simulink model "Cell_Balancer_V_2"  (R2026b)
settings: Solver=VariableStepAuto  StopTime=72000
InitFcn:
  | R=4.2
  | A=.2
  | B=.25
  | C=.24
  | D=.23
  | E=.29
  | F=.22
  | G=.26
  | H=.27
  | I=.28
  | J=.21
libraries: fl_lib x43, nesl_utility x33, batt_lib x10, BatteryCurrentManagement x1
(part 1 of 4)
settings Model: Creator=cbast  LastModifiedBy=cbast
settings SimscapeCC: SimscapeLogType=all  SimscapeNominalValues="[{\"value\":\"1\",\"unit\":\"A\"},{\"value\":\"1\",\"unit\":\"bar\"},{\"value\":\"1\",\"unit\":\"cm^2\"},{\"value\":\"1\",\"unit\":\"cm^3/s\"},{\"value\":\"1\",\"unit\":\"kJ/kg\"},{\"value\":\"1\",\"unit\":\"kW\"},{\"value\":\"1\",\"unit\":\"l\"},{\"value\":\"1\",\"unit\":\"N\"},{\"value\":\"1\",\"unit\":\"N*m\"},{\"value\":\"1\",\"unit\":\"V\"},{\"value\":\"0.001\",\"unit\":\"Wb\"}]"  SimscapeUseEnergyAccounting=off

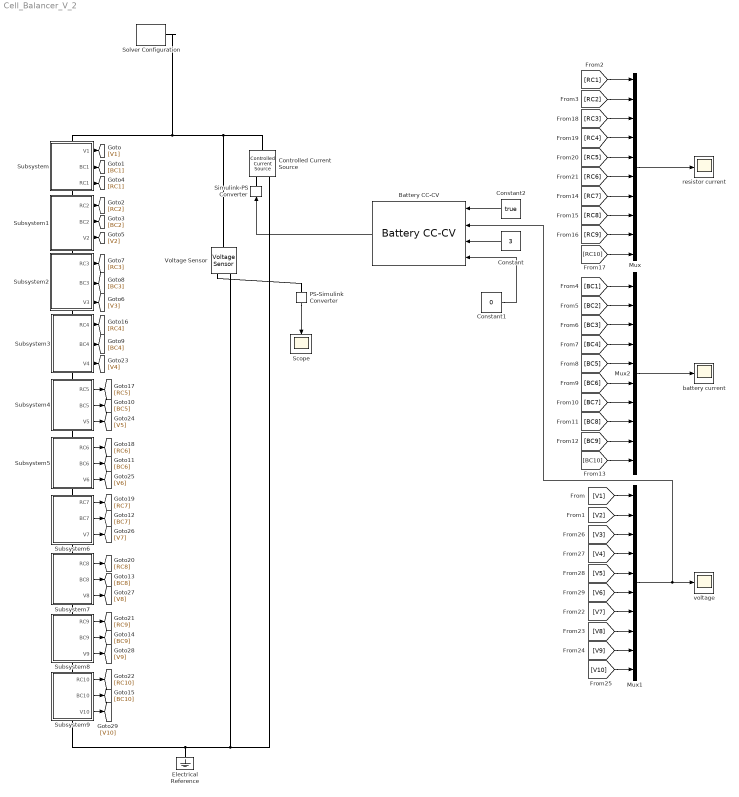
== system Cell_Balancer_V_2 ==
  Battery CC-CV : BatteryCurrentManagement/Battery CC-CV  MinMaxFlag=off  MaxCellVoltage=4.2  Kp=100  Ki=10  Kaw=1  Kt=1  Ts=.1
      settings: LibrarySourceBlock=batt_sl_lib/Current Management/Battery CC-CV
  Constant : Constant  Value=3
  Constant1 : Constant  Value=0
  Constant2 : Constant  Value=true  OutDataTypeStr=boolean
  Controlled Current Source : fl_lib/Electrical/Electrical Sources/Controlled Current Source
  Electrical Reference : fl_lib/Electrical/Electrical Elements/Electrical Reference
  Mux : Mux  Inputs=10
  Mux1 : Mux  Inputs=10
  Mux2 : Mux  Inputs=10
  PS-Simulink Converter : nesl_utility/PS-Simulink Converter  PhysicalDomain=network_engine_domain  SubClassName=ps_output  LeftPortType=input  RightPortType=output  PseudoPeriodic=off  Frequencies=[]  VectorFormat=inherit  Unit=inherit  AffineConversion=off
  Scope : Scope
      settings: ActiveDisplayYMinimum=29.7505090759505  ActiveDisplayYMaximum=43.345712012643816  DataLoggingVariableName=ScopeData3
  Simulink-PS Converter : nesl_utility/Simulink-PS Converter  PhysicalDomain=network_engine_domain  SubClassName=ps_input  LeftPortType=input  RightPortType=output  PseudoPeriodic=off  Frequencies=[]  NoiseDistribution=none  NoiseParameters=[]  Unit=A  AffineConversion=off  FilteringAndDerivatives=provide  SimscapeFilterOrder=1  InputFilterTimeConstant=0.001  UdotUserProvided=0
  Solver Configuration : nesl_utility/Solver Configuration  PhysicalDomain=network_engine_domain  SubClassName=solver  LeftPortType=input  RightPortType=generic  Tones=[]  Harmonics=[]  SimulateNoise=off  Profile=off  UseLocalSampling=off  EnableSwitchedLinearOptims=on  FrequencyDomain=off  UseCCode=off  RelTol=0.001  AbsTol=0.001  MinStep=1e-09  ToWorkspace=off  RevertToSquareIcSolve=off  NumHomotopyIterations=100  PhasorMode=off  PhasorModeNumHarmonics=1  ConsistencySolver=NEWTON_XTOL_AFTER_FTOL  CanonicalOrdering=CANONICAL  OptimizeIntermediates=OPTIMIZED  MulticoreSolverChoice=BACKWARD_EULER  IndexReductionMethod=DerivativeReplacement  DoDC=off  ResidualTolerance=1e-09  ConsistencyTolSource=GLOBAL  ConsistencyAbsTol=0.001  ConsistencyRelTol=0.001  ConsistencyTolFactor=0.001  UseLocalSolver=off  LocalSolverChoice=NE_BACKWARD_EULER_ADVANCER  ResolveIndetEquations=on  FunctionEvalNumThread=1  LocalSolverSampleTime=0.001  DoFixedCost=off  MaxNonlinIter=3  MaxModeIter=2  ComputeImpulses=off  ImpulseIterations=2  LinearAlgebra=auto  LinearAlgebraNumThread=0  EquationFormulation=NE_TIME_EF  DelaysMemoryBudget=1024  AutomaticFiltering=on  FilteringTimeConstant=0.001  PartitionStorageMethod=AS_NEEDED  PartitionMemoryBudget=1024  PartitionMethod=BALANCED  MultibodyUseLocalSolver=off  MultibodyLocalSolverChoice=ODE1  MultibodyLocalSolverSampleTime=0.001
  Subsystem : Subsystem
      settings: PortSchema="{\"entries\":[{\"content\":{\"sides\":[{\"content\":{\"connectorIds\":[\"LConn1\"]},\"type\":\"ConnectorPlacement.EquallySpacedRectSide\",\"uuid\":\"cf979a16-a91b-4829-8e8c-47878ae37a6b\"},{\"content\":{\"connectorIds\":[\"Out1\",\"Out2\",\"Out3\"],\"side\":\"RIGHT\"},\"type\":\"ConnectorPlacement.EquallySpacedRectSide\",\"uuid\":\"6e20e9dd-b02d-4dd9-9bba-83c5ab962d64\"},{\"content\":{\"connectorIds\":[\"LConn2\"],\"side\":\"TOP\"},\"type\":\"ConnectorPlacement.EquallySpacedRectSide\",\"uuid\":\"a7acf913-948b-411d-bbec-040cc670f398\"},{\"content\":{\"connectorIds\":[\"RConn1\"],\"side\":\"BOTTOM\"},\"type\":\"ConnectorPlacement.EquallySpacedRectSide\",\"uuid\":\"1d5d0df0-1bd4-46ff-b3f2-dbc3a67d8787\"}]},\"type\":\"ConnectorPlacement.EquallySpacedConnector\",\"uuid\":\"c3ff8ae8-2df9-499f-8763-7ecb3999170d\"}],\"packageUris\":[\"http://schema.mathworks.com/mf0/Connector/R2020b\"],\"version\":\"1.0\"}"
  Subsystem1 : Subsystem
      settings: PortSchema="{\"entries\":[{\"content\":{\"sides\":[{\"content\":{\"connectorIds\":[\"LConn1\"]},\"type\":\"ConnectorPlacement.EquallySpacedRectSide\",\"uuid\":\"b864f2b2-5928-4e80-8598-6ae066b8b686\"},{\"content\":{\"connectorIds\":[\"Out1\",\"Out2\",\"Out3\"],\"side\":\"RIGHT\"},\"type\":\"ConnectorPlacement.EquallySpacedRectSide\",\"uuid\":\"4c0824a7-ad18-427d-825c-0601e9e3c2a5\"},{\"content\":{\"connectorIds\":[\"LConn2\"],\"side\":\"TOP\"},\"type\":\"ConnectorPlacement.EquallySpacedRectSide\",\"uuid\":\"58eac08c-ab90-4096-8c71-26645031beff\"},{\"content\":{\"connectorIds\":[\"RConn1\"],\"side\":\"BOTTOM\"},\"type\":\"ConnectorPlacement.EquallySpacedRectSide\",\"uuid\":\"928b4b2b-69e3-456a-8822-74aa848d5ef0\"}]},\"type\":\"ConnectorPlacement.EquallySpacedConnector\",\"uuid\":\"d1889de4-d401-4a0f-84af-d9f011bf39d7\"}],\"packageUris\":[\"http://schema.mathworks.com/mf0/Connector/R2020b\"],\"version\":\"1.0\"}"
  Subsystem2 : Subsystem
      settings: PortSchema="{\"entries\":[{\"content\":{\"sides\":[{\"content\":{\"connectorIds\":[\"LConn1\"]},\"type\":\"ConnectorPlacement.EquallySpacedRectSide\",\"uuid\":\"b864f2b2-5928-4e80-8598-6ae066b8b686\"},{\"content\":{\"connectorIds\":[\"Out1\",\"Out2\",\"Out3\"],\"side\":\"RIGHT\"},\"type\":\"ConnectorPlacement.EquallySpacedRectSide\",\"uuid\":\"4c0824a7-ad18-427d-825c-0601e9e3c2a5\"},{\"content\":{\"connectorIds\":[\"LConn2\"],\"side\":\"TOP\"},\"type\":\"ConnectorPlacement.EquallySpacedRectSide\",\"uuid\":\"58eac08c-ab90-4096-8c71-26645031beff\"},{\"content\":{\"connectorIds\":[\"RConn1\"],\"side\":\"BOTTOM\"},\"type\":\"ConnectorPlacement.EquallySpacedRectSide\",\"uuid\":\"928b4b2b-69e3-456a-8822-74aa848d5ef0\"}]},\"type\":\"ConnectorPlacement.EquallySpacedConnector\",\"uuid\":\"d1889de4-d401-4a0f-84af-d9f011bf39d7\"}],\"packageUris\":[\"http://schema.mathworks.com/mf0/Connector/R2020b\"],\"version\":\"1.0\"}"
  Subsystem3 : Subsystem
      settings: PortSchema="{\"entries\":[{\"content\":{\"sides\":[{\"content\":{\"connectorIds\":[\"LConn1\"]},\"type\":\"ConnectorPlacement.EquallySpacedRectSide\",\"uuid\":\"b864f2b2-5928-4e80-8598-6ae066b8b686\"},{\"content\":{\"connectorIds\":[\"Out1\",\"Out2\",\"Out3\"],\"side\":\"RIGHT\"},\"type\":\"ConnectorPlacement.EquallySpacedRectSide\",\"uuid\":\"4c0824a7-ad18-427d-825c-0601e9e3c2a5\"},{\"content\":{\"connectorIds\":[\"LConn2\"],\"side\":\"TOP\"},\"type\":\"ConnectorPlacement.EquallySpacedRectSide\",\"uuid\":\"58eac08c-ab90-4096-8c71-26645031beff\"},{\"content\":{\"connectorIds\":[\"RConn1\"],\"side\":\"BOTTOM\"},\"type\":\"ConnectorPlacement.EquallySpacedRectSide\",\"uuid\":\"928b4b2b-69e3-456a-8822-74aa848d5ef0\"}]},\"type\":\"ConnectorPlacement.EquallySpacedConnector\",\"uuid\":\"d1889de4-d401-4a0f-84af-d9f011bf39d7\"}],\"packageUris\":[\"http://schema.mathworks.com/mf0/Connector/R2020b\"],\"version\":\"1.0\"}"
  Subsystem4 : Subsystem
      settings: PortSchema="{\"entries\":[{\"content\":{\"sides\":[{\"content\":{\"connectorIds\":[\"LConn1\"]},\"type\":\"ConnectorPlacement.EquallySpacedRectSide\",\"uuid\":\"b864f2b2-5928-4e80-8598-6ae066b8b686\"},{\"content\":{\"connectorIds\":[\"Out1\",\"Out2\",\"Out3\"],\"side\":\"RIGHT\"},\"type\":\"ConnectorPlacement.EquallySpacedRectSide\",\"uuid\":\"4c0824a7-ad18-427d-825c-0601e9e3c2a5\"},{\"content\":{\"connectorIds\":[\"LConn2\"],\"side\":\"TOP\"},\"type\":\"ConnectorPlacement.EquallySpacedRectSide\",\"uuid\":\"58eac08c-ab90-4096-8c71-26645031beff\"},{\"content\":{\"connectorIds\":[\"RConn1\"],\"side\":\"BOTTOM\"},\"type\":\"ConnectorPlacement.EquallySpacedRectSide\",\"uuid\":\"928b4b2b-69e3-456a-8822-74aa848d5ef0\"}]},\"type\":\"ConnectorPlacement.EquallySpacedConnector\",\"uuid\":\"d1889de4-d401-4a0f-84af-d9f011bf39d7\"}],\"packageUris\":[\"http://schema.mathworks.com/mf0/Connector/R2020b\"],\"version\":\"1.0\"}"
  Subsystem5 : Subsystem
      settings: PortSchema="{\"entries\":[{\"content\":{\"sides\":[{\"content\":{\"connectorIds\":[\"LConn1\"]},\"type\":\"ConnectorPlacement.EquallySpacedRectSide\",\"uuid\":\"b864f2b2-5928-4e80-8598-6ae066b8b686\"},{\"content\":{\"connectorIds\":[\"Out1\",\"Out2\",\"Out3\"],\"side\":\"RIGHT\"},\"type\":\"ConnectorPlacement.EquallySpacedRectSide\",\"uuid\":\"4c0824a7-ad18-427d-825c-0601e9e3c2a5\"},{\"content\":{\"connectorIds\":[\"LConn2\"],\"side\":\"TOP\"},\"type\":\"ConnectorPlacement.EquallySpacedRectSide\",\"uuid\":\"58eac08c-ab90-4096-8c71-26645031beff\"},{\"content\":{\"connectorIds\":[\"RConn1\"],\"side\":\"BOTTOM\"},\"type\":\"ConnectorPlacement.EquallySpacedRectSide\",\"uuid\":\"928b4b2b-69e3-456a-8822-74aa848d5ef0\"}]},\"type\":\"ConnectorPlacement.EquallySpacedConnector\",\"uuid\":\"d1889de4-d401-4a0f-84af-d9f011bf39d7\"}],\"packageUris\":[\"http://schema.mathworks.com/mf0/Connector/R2020b\"],\"version\":\"1.0\"}"
  Subsystem6 : Subsystem
      settings: PortSchema="{\"entries\":[{\"content\":{\"sides\":[{\"content\":{\"connectorIds\":[\"LConn1\"]},\"type\":\"ConnectorPlacement.EquallySpacedRectSide\",\"uuid\":\"b864f2b2-5928-4e80-8598-6ae066b8b686\"},{\"content\":{\"connectorIds\":[\"Out1\",\"Out2\",\"Out3\"],\"side\":\"RIGHT\"},\"type\":\"ConnectorPlacement.EquallySpacedRectSide\",\"uuid\":\"4c0824a7-ad18-427d-825c-0601e9e3c2a5\"},{\"content\":{\"connectorIds\":[\"LConn2\"],\"side\":\"TOP\"},\"type\":\"ConnectorPlacement.EquallySpacedRectSide\",\"uuid\":\"58eac08c-ab90-4096-8c71-26645031beff\"},{\"content\":{\"connectorIds\":[\"RConn1\"],\"side\":\"BOTTOM\"},\"type\":\"ConnectorPlacement.EquallySpacedRectSide\",\"uuid\":\"928b4b2b-69e3-456a-8822-74aa848d5ef0\"}]},\"type\":\"ConnectorPlacement.EquallySpacedConnector\",\"uuid\":\"d1889de4-d401-4a0f-84af-d9f011bf39d7\"}],\"packageUris\":[\"http://schema.mathworks.com/mf0/Connector/R2020b\"],\"version\":\"1.0\"}"
  Subsystem7 : Subsystem
      settings: PortSchema="{\"entries\":[{\"content\":{\"sides\":[{\"content\":{\"connectorIds\":[\"LConn1\"]},\"type\":\"ConnectorPlacement.EquallySpacedRectSide\",\"uuid\":\"b864f2b2-5928-4e80-8598-6ae066b8b686\"},{\"content\":{\"connectorIds\":[\"Out1\",\"Out2\",\"Out3\"],\"side\":\"RIGHT\"},\"type\":\"ConnectorPlacement.EquallySpacedRectSide\",\"uuid\":\"4c0824a7-ad18-427d-825c-0601e9e3c2a5\"},{\"content\":{\"connectorIds\":[\"LConn2\"],\"side\":\"TOP\"},\"type\":\"ConnectorPlacement.EquallySpacedRectSide\",\"uuid\":\"58eac08c-ab90-4096-8c71-26645031beff\"},{\"content\":{\"connectorIds\":[\"RConn1\"],\"side\":\"BOTTOM\"},\"type\":\"ConnectorPlacement.EquallySpacedRectSide\",\"uuid\":\"928b4b2b-69e3-456a-8822-74aa848d5ef0\"}]},\"type\":\"ConnectorPlacement.EquallySpacedConnector\",\"uuid\":\"d1889de4-d401-4a0f-84af-d9f011bf39d7\"}],\"packageUris\":[\"http://schema.mathworks.com/mf0/Connector/R2020b\"],\"version\":\"1.0\"}"
  Subsystem8 : Subsystem
      settings: PortSchema="{\"entries\":[{\"content\":{\"sides\":[{\"content\":{\"connectorIds\":[\"LConn1\"]},\"type\":\"ConnectorPlacement.EquallySpacedRectSide\",\"uuid\":\"b864f2b2-5928-4e80-8598-6ae066b8b686\"},{\"content\":{\"connectorIds\":[\"Out1\",\"Out2\",\"Out3\"],\"side\":\"RIGHT\"},\"type\":\"ConnectorPlacement.EquallySpacedRectSide\",\"uuid\":\"4c0824a7-ad18-427d-825c-0601e9e3c2a5\"},{\"content\":{\"connectorIds\":[\"LConn2\"],\"side\":\"TOP\"},\"type\":\"ConnectorPlacement.EquallySpacedRectSide\",\"uuid\":\"58eac08c-ab90-4096-8c71-26645031beff\"},{\"content\":{\"connectorIds\":[\"RConn1\"],\"side\":\"BOTTOM\"},\"type\":\"ConnectorPlacement.EquallySpacedRectSide\",\"uuid\":\"928b4b2b-69e3-456a-8822-74aa848d5ef0\"}]},\"type\":\"ConnectorPlacement.EquallySpacedConnector\",\"uuid\":\"d1889de4-d401-4a0f-84af-d9f011bf39d7\"}],\"packageUris\":[\"http://schema.mathworks.com/mf0/Connector/R2020b\"],\"version\":\"1.0\"}"
  Subsystem9 : Subsystem
      settings: PortSchema="{\"entries\":[{\"content\":{\"sides\":[{\"content\":{\"connectorIds\":[\"LConn1\"]},\"type\":\"ConnectorPlacement.EquallySpacedRectSide\",\"uuid\":\"b864f2b2-5928-4e80-8598-6ae066b8b686\"},{\"content\":{\"connectorIds\":[\"Out1\",\"Out2\",\"Out3\"],\"side\":\"RIGHT\"},\"type\":\"ConnectorPlacement.EquallySpacedRectSide\",\"uuid\":\"4c0824a7-ad18-427d-825c-0601e9e3c2a5\"},{\"content\":{\"connectorIds\":[\"LConn2\"],\"side\":\"TOP\"},\"type\":\"ConnectorPlacement.EquallySpacedRectSide\",\"uuid\":\"58eac08c-ab90-4096-8c71-26645031beff\"},{\"content\":{\"connectorIds\":[\"RConn1\"],\"side\":\"BOTTOM\"},\"type\":\"ConnectorPlacement.EquallySpacedRectSide\",\"uuid\":\"928b4b2b-69e3-456a-8822-74aa848d5ef0\"}]},\"type\":\"ConnectorPlacement.EquallySpacedConnector\",\"uuid\":\"d1889de4-d401-4a0f-84af-d9f011bf39d7\"}],\"packageUris\":[\"http://schema.mathworks.com/mf0/Connector/R2020b\"],\"version\":\"1.0\"}"
  Voltage Sensor : fl_lib/Electrical/Electrical Sensors/Voltage Sensor
  battery current : Scope
      settings: ActiveDisplayYMinimum=-0.32310664048068816  ActiveDisplayYMaximum=2.5809557460332671  DataLoggingVariableName=ScopeData2
  resistor current : Scope
      settings: ActiveDisplayYMinimum=0.68694599163620873  ActiveDisplayYMaximum=1.0369030277450046
  voltage : Scope
      settings: ActiveDisplayYMinimum=2.8851731648720769  ActiveDisplayYMaximum=4.3549927165290168
  wires:
  Mux/1 -> resistor current/1
  Mux1/1 -> Battery CC-CV/2, voltage/1
  [BC2] -> Mux2/2
  [BC1] -> Mux2/1
  Mux2/1 -> battery current/1
  [RC1] -> Mux/1
  [RC2] -> Mux/2
  [V2] -> Mux1/2
  [V1] -> Mux1/1
  Subsystem/1(V1) -> [V1]
  Subsystem/2(BC1) -> [BC1]
  Subsystem/3(RC1) -> [RC1]
  Subsystem1/1(RC2) -> [RC2]
  Subsystem1/2(BC2) -> [BC2]
  Subsystem1/3(V2) -> [V2]
  [BC3] -> Mux2/3
  [BC4] -> Mux2/4
  [BC5] -> Mux2/5
  [BC6] -> Mux2/6
  [BC7] -> Mux2/7
  [BC8] -> Mux2/8
  [BC9] -> Mux2/9
  [BC10] -> Mux2/10
  [RC5] -> Mux/5
  [RC4] -> Mux/4
  [RC6] -> Mux/6
  [RC10] -> Mux/10
  [RC9] -> Mux/9
  [RC8] -> Mux/8
  [RC7] -> Mux/7
  [V3] -> Mux1/3
  [V4] -> Mux1/4
  [V5] -> Mux1/5
  [V6] -> Mux1/6
  [V7] -> Mux1/7
  [V8] -> Mux1/8
  [V9] -> Mux1/9
  [V10] -> Mux1/10
  Subsystem2/3(V3) -> [V3]
  Subsystem2/2(BC3) -> [BC3]
  Subsystem2/1(RC3) -> [RC3]
  Subsystem3/2(BC4) -> [BC4]
  Subsystem5/2(BC6) -> [BC6]
  Subsystem3/1(RC4) -> [RC4]
  Subsystem4/1(RC5) -> [RC5]
  Subsystem4/2(BC5) -> [BC5]
  Subsystem3/3(V4) -> [V4]
  Subsystem4/3(V5) -> [V5]
  Subsystem5/1(RC6) -> [RC6]
  Subsystem5/3(V6) -> [V6]
  Subsystem6/1(RC7) -> [RC7]
  Subsystem6/2(BC7) -> [BC7]
  Subsystem7/3(V8) -> [V8]
  Subsystem8/3(V9) -> [V9]
  Subsystem7/2(BC8) -> [BC8]
  Subsystem7/1(RC8) -> [RC8]
  Subsystem6/3(V7) -> [V7]
  Subsystem8/1(RC9) -> [RC9]
  Subsystem8/2(BC9) -> [BC9]
  Subsystem9/1(RC10) -> [RC10]
  Subsystem9/2(BC10) -> [BC10]
  Subsystem9/3(V10) -> [V10]
  [RC3] -> Mux/3
  PS-Simulink Converter/1 -> Scope/1
  Battery CC-CV/1 -> Simulink-PS Converter/1
  Constant/1 -> Battery CC-CV/3
  Constant1/1 -> Battery CC-CV/4
  Constant2/1 -> Battery CC-CV/1
  connections:
  Simulink-PS Converter/RConn1 -- Controlled Current Source/RConn1
  Solver Configuration/RConn1 -- Controlled Current Source/LConn1 -- Voltage Sensor/LConn1 -- Subsystem/LConn2
  Controlled Current Source/RConn2 -- Subsystem9/RConn1 -- Electrical Reference/LConn1 -- Voltage Sensor/RConn2
  Subsystem/RConn1 -- Subsystem1/LConn2
  Subsystem2/LConn2 -- Subsystem1/RConn1
  Subsystem3/LConn2 -- Subsystem2/RConn1
  Subsystem4/LConn2 -- Subsystem3/RConn1
  Subsystem5/LConn2 -- Subsystem4/RConn1
  Subsystem6/LConn2 -- Subsystem5/RConn1
  Subsystem7/LConn2 -- Subsystem6/RConn1
  Subsystem8/LConn2 -- Subsystem7/RConn1
  Subsystem9/LConn2 -- Subsystem8/RConn1
  PS-Simulink Converter/LConn1 -- Voltage Sensor/RConn1

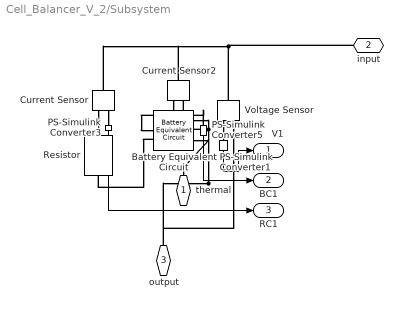
== system Cell_Balancer_V_2/Subsystem ==
  Battery Equivalent Circuit : batt_lib/Cells/Battery Equivalent Circuit  BatteryCapacity=3 A*hr  ThermalModel=simscape.battery.enum.cells.BatteryThermalModel.LumpedThermalMass  ExtrapolationMethod=simscape.enum.extrapolation.nearest  SOCBreakpoints=[0, .1, .25, .5, .75, .9, 1]  TemperatureBreakpoints=[278, 293, 313] K  OpenCircuitVoltage=[3.5057, 3.566, 3.6337, 3.7127, 3.9259, 4.0777, 4.1928] V  OpenCircuitVoltageThermal=|  VoltageRange=[0, inf] V  HysteresisModel=simscape.battery.enum.cells.HysteresisModel.none  MaximumHysteresisVoltage=[0, 0, 0, 0, 0, 0, 0] V  InstantaneousHysteresisVoltage=[0, 0, 0, 0, 0, 0, 0] V  HysteresisRate=0.1  MaximumHysteresisVoltageThermal=[0, 0, 0; 0, 0, 0; 0, 0, 0; 0, 0, 0; 0, 0, 0; 0, 0, 0; 0, 0, 0] V  InstantaneousHysteresisVoltageThermal=[0, 0, 0; 0, 0, 0; 0, 0, 0; 0, 0, 0; 0, 0, 0; 0, 0, 0; 0, 0, 0] V  HysteresisRateThermal=0.1  ResistanceSOCBreakpoints=[0, .1, .25, .5, .75, .9, 1]  ResistanceTemperatureBreakpoints=[278, 293, 313] K  ResistanceCurrentBreakpoints=[-1, 0, 1] A  CurrentDependence=simscape.battery.enum.cells.CurrentDependence.Disabled  R0=[.0085, .0085, .0087, .0082, .0083, .0085, .0085] Ohm  R0I=[.0117, .0085, .009; .011, .0085, .009; .0114, .0087, .0092; .0107, .0082, .0088; .0107, .0083, .0091; .0113, .0085, .0089; .0116, .0085, .0089] Ohm  R0Thermal=[.0117, .0085, .009; .011, .0085, .009; .0114, .0087, .0092; .0107, .0082, .0088; .0107, .0083, .0091; .0113, .0085, .0089; .0116, .0085, .0089] Ohm  R0ThermalI=repmat([.0117, .0085, .009; .011, .0085, .009; .0114, .0087, .0092; .0107, .0082, .0088; .0107, .0083, .0091; .0113, .0085, .0089; .0116, .0085, .0089], 1, 1, 3) Ohm  DischargeR0=[.0085, .0085, .0087, .0082, .0083, .0085, .0085] Ohm  ChargeR0=[.0085, .0085, .0087, .0082, .0083, .0085, .0085] Ohm  ChargeR0Thermal=[.0117, .0085, .009; .011, .0085, .009; .0114, .0087, .0092; .0107, .0082, .0088; .0107, .0083, .0091; .0113, .0085, .0089; .0116, .0085, .0089] Ohm  DischargeR0Thermal=[.0117, .0085, .009; .011, .0085, .009; .0114, .0087, .0092; .0107, .0082, .0088; .0107, .0083, .0091; .0113, .0085, .0089; .0116, .0085, .0089] Ohm  RCPairs=simscape.battery.enum.cells.RCPairs.noDynamics  R1=[.0029, .0024, .0026, .0016, .0023, .0018, .0017] Ohm  Tau1=[36, 45, 105, 29, 77, 33, 39] s  R2=[.0029, .0024, .0026, .0016, .0023, .0018, .0017] Ohm  Tau2=[36, 45, 105, 29, 77, 33, 39] s  R3=[.0029, .0024, .0026, .0016, .0023, .0018, .0017] Ohm  Tau3=[36, 45, 105, 29, 77, 33, 39] s  R1I=[.0109, .0029, .0013; .0069, .0024, .0012; .0047, .0026, .0013; .0034, .0016, .001; .0033, .0023, .0014; .0033, .0018, .0011; .0028, .0017, .0011] Ohm  Tau1I=[20, 36, 39; 31, 45, 39; 109, 105, 61; 36, 29, 26; 59, 77, 67; 40, 33, 29; 25, 39, 33] s  R2I=[.0109, .0029, .0013; .0069, .0024, .0012; .0047, .0026, .0013; .0034, .0016, .001; .0033, .0023, .0014; .0033, .0018, .0011; .0028, .0017, .0011] Ohm  Tau2I=[20, 36, 39; 31, 45, 39; 109, 105, 61; 36, 29, 26; 59, 77, 67; 40, 33, 29; 25, 39, 33] s  R3I=[.0109, .0029, .0013; .0069, .0024, .0012; .0047, .0026, .0013; .0034, .0016, .001; .0033, .0023, .0014; .0033, .0018, .0011; .0028, .0017, .0011] Ohm  Tau3I=[20, 36, 39; 31, 45, 39; 109, 105, 61; 36, 29, 26; 59, 77, 67; 40, 33, 29; 25, 39, 33] s  DischargeR1=[.0029, .0024, .0026, .0016, .0023, .0018, .0017] Ohm  DischargeTau1=[36, 45, 105, 29, 77, 33, 39] s  ChargeR1=[.0029, .0024, .0026, .0016, .0023, .0018, .0017] Ohm  ChargeTau1=[36, 45, 105, 29, 77, 33, 39] s  DischargeR2=[.0029, .0024, .0026, .0016, .0023, .0018, .0017] Ohm  DischargeTau2=[36, 45, 105, 29, 77, 33, 39] s  ChargeR2=[.0029, .0024, .0026, .0016, .0023, .0018, .0017] Ohm  ChargeTau2=[36, 45, 105, 29, 77, 33, 39] s  DischargeR3=[.0029, .0024, .0026, .0016, .0023, .0018, .0017] Ohm  DischargeTau3=[36, 45, 105, 29, 77, 33, 39] s  ChargeR3=[.0029, .0024, .0026, .0016, .0023, .0018, .0017] Ohm  ChargeTau3=[36, 45, 105, 29, 77, 33, 39] s  R1Thermal=[.0109, .0029, .0013; .0069, .0024, .0012; .0047, .0026, .0013; .0034, .0016, .001; .0033, .0023, .0014; .0033, .0018, .0011; .0028, .0017, .0011] Ohm  Tau1Thermal=[20, 36, 39; 31, 45, 39; 109, 105, 61; 36, 29, 26; 59, 77, 67; 40, 33, 29; 25, 39, 33] s  R2Thermal=[.0109, .0029, .0013; .0069, .0024, .0012; .0047, .0026, .0013; .0034, .0016, .001; .0033, .0023, .0014; .0033, .0018, .0011; .0028, .0017, .0011] Ohm  Tau2Thermal=[20, 36, 39; 31, 45, 39; 109, 105, 61; 36, 29, 26; 59, 77, 67; 40, 33, 29; 25, 39, 33] s  R3Thermal=[.0109, .0029, .0013; .0069, .0024, .0012; .0047, .0026, .0013; .0034, .0016, .001; .0033, .0023, .0014; .0033, .0018, .0011; .0028, .0017, .0011] Ohm  Tau3Thermal=[20, 36, 39; 31, 45, 39; 109, 105, 61; 36, 29, 26; 59, 77, 67; 40, 33, 29; 25, 39, 33] s  R1ThermalI=repmat([.0109, .0029, .0013; .0069, .0024, .0012; .0047, .0026, .0013; .0034, .0016, .001; .0033, .0023, .0014; .0033, .0018, .0011; .0028, .0017, .0011], 1, 1, 3) Ohm  Tau1ThermalI=repmat([20, 36, 39; 31, 45, 39; 109, 105, 61; 36, 29, 26; 59, 77, 67; 40, 33, 29; 25, 39, 33], 1, 1, 3) s  R2ThermalI=repmat([.0109, .0029, .0013; .0069, .0024, .0012; .0047, .0026, .0013; .0034, .0016, .001; .0033, .0023, .0014; .0033, .0018, .0011; .0028, .0017, .0011], 1, 1, 3) Ohm  Tau2ThermalI=repmat([20, 36, 39; 31, 45, 39; 109, 105, 61; 36, 29, 26; 59, 77, 67; 40, 33, 29; 25, 39, 33], 1, 1, 3) s  R3ThermalI=repmat([.0109, .0029, .0013; .0069, .0024, .0012; .0047, .0026, .0013; .0034, .0016, .001; .0033, .0023, .0014; .0033, .0018, .0011; .0028, .0017, .0011], 1, 1, 3) Ohm  Tau3ThermalI=repmat([20, 36, 39; 31, 45, 39; 109, 105, 61; 36, 29, 26; 59, 77, 67; 40, 33, 29; 25, 39, 33], 1, 1, 3) s  DischargeR1Thermal=[.0109, .0029, .0013; .0069, .0024, .0012; .0047, .0026, .0013; .0034, .0016, .001; .0033, .0023, .0014; .0033, .0018, .0011; .0028, .0017, .0011] Ohm  DischargeTau1Thermal=[20, 36, 39; 31, 45, 39; 109, 105, 61; 36, 29, 26; 59, 77, 67; 40, 33, 29; 25, 39, 33] s  ChargeR1Thermal=[.0109, .0029, .0013; .0069, .0024, .0012; .0047, .0026, .0013; .0034, .0016, .001; .0033, .0023, .0014; .0033, .0018, .0011; .0028, .0017, .0011] Ohm  ChargeTau1Thermal=[20, 36, 39; 31, 45, 39; 109, 105, 61; 36, 29, 26; 59, 77, 67; 40, 33, 29; 25, 39, 33] s  DischargeR2Thermal=[.0109, .0029, .0013; .0069, .0024, .0012; .0047, .0026, .0013; .0034, .0016, .001; .0033, .0023, .0014; .0033, .0018, .0011; .0028, .0017, .0011] Ohm  DischargeTau2Thermal=[20, 36, 39; 31, 45, 39; 109, 105, 61; 36, 29, 26; 59, 77, 67; 40, 33, 29; 25, 39, 33] s  ChargeR2Thermal=[.0109, .0029, .0013; .0069, .0024, .0012; .0047, .0026, .0013; .0034, .0016, .001; .0033, .0023, .0014; .0033, .0018, .0011; .0028, .0017, .0011] Ohm  ChargeTau2Thermal=[20, 36, 39; 31, 45, 39; 109, 105, 61; 36, 29, 26; 59, 77, 67; 40, 33, 29; 25, 39, 33] s  DischargeR3Thermal=[.0109, .0029, .0013; .0069, .0024, .0012; .0047, .0026, .0013; .0034, .0016, .001; .0033, .0023, .0014; .0033, .0018, .0011; .0028, .0017, .0011] Ohm  DischargeTau3Thermal=[20, 36, 39; 31, 45, 39; 109, 105, 61; 36, 29, 26; 59, 77, 67; 40, 33, 29; 25, 39, 33] s  ChargeR3Thermal=[.0109, .0029, .0013; .0069, .0024, .0012; .0047, .0026, .0013; .0034, .0016, .001; .0033, .0023, .0014; .0033, .0018, .0011; .0028, .0017, .0011] Ohm  ChargeTau3Thermal=[20, 36, 39; 31, 45, 39; 109, 105, 61; 36, 29, 26; 59, 77, 67; 40, 33, 29; 25, 39, 33] s  SelfDischargeResistor=simscape.battery.enum.cells.BatteryEnable.Disabled  SelfDischargeR=7e3 Ohm  SelfDischargeRThermal=[8000, 7000, 6000] Ohm  CyclingAgingMethod=simscape.battery.enum.cells.CyclingAgingMethod.disabled  CycleCalculationMethod=simscape.battery.enum.cells.CycleCalculationMethod.EquivalentCycles  NumDisCycles=100  OCVChange=0  R0Change=0  CapacityChange=0  SelfDischargeRChange=0  R1Change=0  R2Change=0  R3Change=0  NumDisCyclesBreakpoints=[0, 100, 200, 300]  AgingTemperatureBreakpoints=[298.15, 323.15] K  AgingCurrentBreakpoints=[-.1, -.5, -5] A  OCVChangeVec=[0, 0, 0, 0]  OCVChangeThermal=[0, 0; 0, 0; 0, 0; 0, 0]  R0ChangeVec=[0, 0, 0, 0]  R0ChangeThermal=[0, 0; 0, 0; 0, 0; 0, 0]  R0ChangeThermalI=repmat(0, 4, 2, 3)  R0CyclingChangeInitialTarget=0  CapacityChangeVec=[0, 0, 0, 0]  CapacityChangeThermal=[0, 0; 0, 0; 0, 0; 0, 0]  CapacityChangeThermalI=repmat(0, 4, 2, 3)  CapacityCyclingChangeInitialTarget=0  SelfDischargeRChangeVec=[0, 0, 0, 0]  SelfDischargeRChangeThermal=[0, 0; 0, 0; 0, 0; 0, 0]  SelfDischargeRChangeThermalI=repmat(0, 4, 2, 3)  SelfDischargeRCyclingChangeInitialTarget=0  R1ChangeVec=[0, 0, 0, 0]  R1ChangeThermal=[0, 0; 0, 0; 0, 0; 0, 0]  R1ChangeThermalI=repmat(0, 4, 2, 3)  R1CyclingChangeInitialTarget=0  R2ChangeVec=[0, 0, 0, 0]  R2ChangeThermal=[0, 0; 0, 0; 0, 0; 0, 0]  R2ChangeThermalI=repmat(0, 4, 2, 3)  R2CyclingChangeInitialTarget=0  R3ChangeVec=[0, 0, 0, 0]  R3ChangeThermal=[0, 0; 0, 0; 0, 0; 0, 0]  R3ChangeThermalI=repmat(0, 4, 2, 3)  R3CyclingChangeInitialTarget=0  CalendarAgeResistance=simscape.battery.enum.cells.BatteryEnable.Disabled  CalendarAgeCapacity=simscape.battery.enum.cells.BatteryEnable.Disabled  CalendarAgingMethod=simscape.battery.enum.cells.CalendarAgingMethod.equation  StorageVariable=simscape.battery.enum.cells.StorageVariable.OCV  OCVDuringStorage=0.9  SOCDuringStorage=0.6  StorageTimeIntervals=[0] d  StorageTemperatures=[273] K  ResistanceScalingOCV=2.2134e6  ResistanceScalingOCVOffset=1.632e6  ResistanceExponentialIncrease=0.515833569 V  ResistanceTimeExponent=0.75  ResistanceAgeTemperatureBreakpoints=[273.15, 298.15, 323.15] K  ResistanceAgeTimeBreakpoints=[0, 90, 180, 270] d  PercentResistanceChange=[0, 0, 0]  ResistanceTimeBreakpoints=100 d  PercentResistanceChangeThermal=[0, 0, 0; 0, 0, 0; 0, 0, 0; 0, 0, 0]  CapacityScalingOCV=1.5097e07  CapacityScalingOCVOffset=8.3625e06  CapacityExponentialIncrease=0.6011 V  CapacityTimeExponent=0.75  CapacityAgeTemperatureBreakpoints=[273.15, 298.15, 323.15] K  CapacityAgeTimeBreakpoints=[0, 90, 180, 270] d  PercentCapacityChange=[0, 0, 0]  CapacityTimeBreakpoints=100 d  PercentCapacityChangeThermal=[0, 0, 0; 0, 0, 0; 0, 0, 0; 0, 0, 0]  SimulationTemperature=298.15 K  BatteryThermalMass=100 J/K  NumThermalModels=6  ThermalConductivityZ=18 W/(K*m)  CrossSectionalAreaXY=3.5e-4 m^2  Height=0.07 m  ReversibleHeatModel=simscape.battery.enum.cells.ReversibleHeatModel.Disabled  EntropicCoefficient=[0, 0, 0, 0, 0, 0, 0] mV/K  CurrentDirectionality=simscape.battery.enum.cells.BatteryEnable.Disabled  stateOfCharge_specify=on  stateOfCharge_priority=High  stateOfCharge=A  stateOfCharge_nominal_specify=off  stateOfCharge_nominal_value=1  stateOfCharge_nominal_unit=1  batteryVoltage_specify=off  batteryVoltage_priority=None  batteryVoltage=0 V  batteryVoltage_nominal_specify=off  batteryVoltage_nominal_value=1  batteryVoltage_nominal_unit=V  batteryCurrent_specify=off  batteryCurrent_priority=None  batteryCurrent=0 A  batteryCurrent_nominal_specify=off  batteryCurrent_nominal_value=1  batteryCurrent_nominal_unit=A  numCycles_specify=off  numCycles_priority=High  numCycles=0  numCycles_nominal_specify=off  numCycles_nominal_value=1  numCycles_nominal_unit=1  batteryTemperature_specify=off  batteryTemperature_priority=High  batteryTemperature=298.15 K  batteryTemperature_nominal_specify=off  batteryTemperature_nominal_value=1  batteryTemperature_nominal_unit=K  hysteresisState_specify=off  hysteresisState_priority=High  hysteresisState=0  hysteresisState_nominal_specify=off  hysteresisState_nominal_value=1  hysteresisState_nominal_unit=1  isExothermFaulted_specify=off  isExothermFaulted_priority=None  isExothermFaulted=0  isExothermFaulted_nominal_specify=off  isExothermFaulted_nominal_value=1  isExothermFaulted_nominal_unit=1  reactionHeatRate_specify=off  reactionHeatRate_priority=None  reactionHeatRate=0 W  reactionHeatRate_nominal_specify=off  reactionHeatRate_nominal_value=1  reactionHeatRate_nominal_unit=W  reactionExtent_specify=off  reactionExtent_priority=None  reactionExtent=0  reactionExtent_nominal_specify=off  reactionExtent_nominal_value=1  reactionExtent_nominal_unit=1  shortResistorPower_specify=off  shortResistorPower_priority=None  shortResistorPower=0 W  shortResistorPower_nominal_specify=off  shortResistorPower_nominal_value=1  shortResistorPower_nominal_unit=W
      | [
      |     2.50  2.51  2.52
      |     2.78  2.79  2.80
      |     3.07  3.08  3.09
      |     3.35  3.36  3.37
      |     3.63  3.64  3.65
      |     3.91  3.92  3.93
      |     4.20  4.21  4.22
      | ]
      |  V
  Current Sensor : fl_lib/Electrical/Electrical Sensors/Current Sensor
  Current Sensor2 : fl_lib/Electrical/Electrical Sensors/Current Sensor
  PS-Simulink Converter1 : nesl_utility/PS-Simulink Converter  PhysicalDomain=network_engine_domain  SubClassName=ps_output  LeftPortType=input  RightPortType=output  PseudoPeriodic=off  Frequencies=[]  VectorFormat=inherit  Unit=inherit  AffineConversion=off
  PS-Simulink Converter3 : nesl_utility/PS-Simulink Converter  PhysicalDomain=network_engine_domain  SubClassName=ps_output  LeftPortType=input  RightPortType=output  PseudoPeriodic=off  Frequencies=[]  VectorFormat=inherit  Unit=inherit  AffineConversion=off
  PS-Simulink Converter5 : nesl_utility/PS-Simulink Converter  PhysicalDomain=network_engine_domain  SubClassName=ps_output  LeftPortType=input  RightPortType=output  PseudoPeriodic=off  Frequencies=[]  VectorFormat=inherit  Unit=inherit  AffineConversion=off
  Resistor : fl_lib/Electrical/Electrical Elements/Resistor  R=R Ohm  i_specify=off  i_priority=None  i=0 A  i_nominal_specify=off  i_nominal_value=1  i_nominal_unit=A  v_specify=off  v_priority=None  v=0 V  v_nominal_specify=off  v_nominal_value=1  v_nominal_unit=V
  Voltage Sensor : fl_lib/Electrical/Electrical Sensors/Voltage Sensor
  thermal : PMIOPort  Side=Left
  input : PMIOPort  Port=2  Side=Left
  output : PMIOPort  Port=3  Side=Right
  V1 : Outport
  BC1 : Outport  Port=2
  RC1 : Outport  Port=3
  wires:
  PS-Simulink Converter1/1 -> V1/1
  PS-Simulink Converter5/1 -> BC1/1
  PS-Simulink Converter3/1 -> RC1/1
  connections:
  Battery Equivalent Circuit/RConn2 -- thermal/RConn1
  Current Sensor2/RConn2 -- Battery Equivalent Circuit/LConn1
  Current Sensor/RConn1 -- PS-Simulink Converter3/LConn1
  Voltage Sensor/RConn1 -- PS-Simulink Converter1/LConn1
  Current Sensor/RConn2 -- Resistor/LConn1
  Current Sensor2/LConn1 -- Current Sensor/LConn1 -- input/RConn1 -- Voltage Sensor/LConn1
  PS-Simulink Converter5/LConn1 -- Current Sensor2/RConn1
  Battery Equivalent Circuit/RConn1 -- Voltage Sensor/RConn2 -- output/RConn1 -- Resistor/RConn1

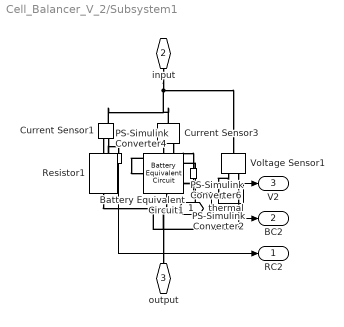
== system Cell_Balancer_V_2/Subsystem1 ==
  Battery Equivalent Circuit1 : batt_lib/Cells/Battery Equivalent Circuit  BatteryCapacity=3 A*hr  ThermalModel=simscape.battery.enum.cells.BatteryThermalModel.LumpedThermalMass  ExtrapolationMethod=simscape.enum.extrapolation.nearest  SOCBreakpoints=[0, .1, .25, .5, .75, .9, 1]  TemperatureBreakpoints=[278, 293, 313] K  OpenCircuitVoltage=[3.5057, 3.566, 3.6337, 3.7127, 3.9259, 4.0777, 4.1928] V  OpenCircuitVoltageThermal=|  VoltageRange=[0, inf] V  HysteresisModel=simscape.battery.enum.cells.HysteresisModel.none  MaximumHysteresisVoltage=[0, 0, 0, 0, 0, 0, 0] V  InstantaneousHysteresisVoltage=[0, 0, 0, 0, 0, 0, 0] V  HysteresisRate=0.1  MaximumHysteresisVoltageThermal=[0, 0, 0; 0, 0, 0; 0, 0, 0; 0, 0, 0; 0, 0, 0; 0, 0, 0; 0, 0, 0] V  InstantaneousHysteresisVoltageThermal=[0, 0, 0; 0, 0, 0; 0, 0, 0; 0, 0, 0; 0, 0, 0; 0, 0, 0; 0, 0, 0] V  HysteresisRateThermal=0.1  ResistanceSOCBreakpoints=[0, .1, .25, .5, .75, .9, 1]  ResistanceTemperatureBreakpoints=[278, 293, 313] K  ResistanceCurrentBreakpoints=[-1, 0, 1] A  CurrentDependence=simscape.battery.enum.cells.CurrentDependence.Disabled  R0=[.0085, .0085, .0087, .0082, .0083, .0085, .0085] Ohm  R0I=[.0117, .0085, .009; .011, .0085, .009; .0114, .0087, .0092; .0107, .0082, .0088; .0107, .0083, .0091; .0113, .0085, .0089; .0116, .0085, .0089] Ohm  R0Thermal=[.0117, .0085, .009; .011, .0085, .009; .0114, .0087, .0092; .0107, .0082, .0088; .0107, .0083, .0091; .0113, .0085, .0089; .0116, .0085, .0089] Ohm  R0ThermalI=repmat([.0117, .0085, .009; .011, .0085, .009; .0114, .0087, .0092; .0107, .0082, .0088; .0107, .0083, .0091; .0113, .0085, .0089; .0116, .0085, .0089], 1, 1, 3) Ohm  DischargeR0=[.0085, .0085, .0087, .0082, .0083, .0085, .0085] Ohm  ChargeR0=[.0085, .0085, .0087, .0082, .0083, .0085, .0085] Ohm  ChargeR0Thermal=[.0117, .0085, .009; .011, .0085, .009; .0114, .0087, .0092; .0107, .0082, .0088; .0107, .0083, .0091; .0113, .0085, .0089; .0116, .0085, .0089] Ohm  DischargeR0Thermal=[.0117, .0085, .009; .011, .0085, .009; .0114, .0087, .0092; .0107, .0082, .0088; .0107, .0083, .0091; .0113, .0085, .0089; .0116, .0085, .0089] Ohm  RCPairs=simscape.battery.enum.cells.RCPairs.noDynamics  R1=[.0029, .0024, .0026, .0016, .0023, .0018, .0017] Ohm  Tau1=[36, 45, 105, 29, 77, 33, 39] s  R2=[.0029, .0024, .0026, .0016, .0023, .0018, .0017] Ohm  Tau2=[36, 45, 105, 29, 77, 33, 39] s  R3=[.0029, .0024, .0026, .0016, .0023, .0018, .0017] Ohm  Tau3=[36, 45, 105, 29, 77, 33, 39] s  R1I=[.0109, .0029, .0013; .0069, .0024, .0012; .0047, .0026, .0013; .0034, .0016, .001; .0033, .0023, .0014; .0033, .0018, .0011; .0028, .0017, .0011] Ohm  Tau1I=[20, 36, 39; 31, 45, 39; 109, 105, 61; 36, 29, 26; 59, 77, 67; 40, 33, 29; 25, 39, 33] s  R2I=[.0109, .0029, .0013; .0069, .0024, .0012; .0047, .0026, .0013; .0034, .0016, .001; .0033, .0023, .0014; .0033, .0018, .0011; .0028, .0017, .0011] Ohm  Tau2I=[20, 36, 39; 31, 45, 39; 109, 105, 61; 36, 29, 26; 59, 77, 67; 40, 33, 29; 25, 39, 33] s  R3I=[.0109, .0029, .0013; .0069, .0024, .0012; .0047, .0026, .0013; .0034, .0016, .001; .0033, .0023, .0014; .0033, .0018, .0011; .0028, .0017, .0011] Ohm  Tau3I=[20, 36, 39; 31, 45, 39; 109, 105, 61; 36, 29, 26; 59, 77, 67; 40, 33, 29; 25, 39, 33] s  DischargeR1=[.0029, .0024, .0026, .0016, .0023, .0018, .0017] Ohm  DischargeTau1=[36, 45, 105, 29, 77, 33, 39] s  ChargeR1=[.0029, .0024, .0026, .0016, .0023, .0018, .0017] Ohm  ChargeTau1=[36, 45, 105, 29, 77, 33, 39] s  DischargeR2=[.0029, .0024, .0026, .0016, .0023, .0018, .0017] Ohm  DischargeTau2=[36, 45, 105, 29, 77, 33, 39] s  ChargeR2=[.0029, .0024, .0026, .0016, .0023, .0018, .0017] Ohm  ChargeTau2=[36, 45, 105, 29, 77, 33, 39] s  DischargeR3=[.0029, .0024, .0026, .0016, .0023, .0018, .0017] Ohm  DischargeTau3=[36, 45, 105, 29, 77, 33, 39] s  ChargeR3=[.0029, .0024, .0026, .0016, .0023, .0018, .0017] Ohm  ChargeTau3=[36, 45, 105, 29, 77, 33, 39] s  R1Thermal=[.0109, .0029, .0013; .0069, .0024, .0012; .0047, .0026, .0013; .0034, .0016, .001; .0033, .0023, .0014; .0033, .0018, .0011; .0028, .0017, .0011] Ohm  Tau1Thermal=[20, 36, 39; 31, 45, 39; 109, 105, 61; 36, 29, 26; 59, 77, 67; 40, 33, 29; 25, 39, 33] s  R2Thermal=[.0109, .0029, .0013; .0069, .0024, .0012; .0047, .0026, .0013; .0034, .0016, .001; .0033, .0023, .0014; .0033, .0018, .0011; .0028, .0017, .0011] Ohm  Tau2Thermal=[20, 36, 39; 31, 45, 39; 109, 105, 61; 36, 29, 26; 59, 77, 67; 40, 33, 29; 25, 39, 33] s  R3Thermal=[.0109, .0029, .0013; .0069, .0024, .0012; .0047, .0026, .0013; .0034, .0016, .001; .0033, .0023, .0014; .0033, .0018, .0011; .0028, .0017, .0011] Ohm  Tau3Thermal=[20, 36, 39; 31, 45, 39; 109, 105, 61; 36, 29, 26; 59, 77, 67; 40, 33, 29; 25, 39, 33] s  R1ThermalI=repmat([.0109, .0029, .0013; .0069, .0024, .0012; .0047, .0026, .0013; .0034, .0016, .001; .0033, .0023, .0014; .0033, .0018, .0011; .0028, .0017, .0011], 1, 1, 3) Ohm  Tau1ThermalI=repmat([20, 36, 39; 31, 45, 39; 109, 105, 61; 36, 29, 26; 59, 77, 67; 40, 33, 29; 25, 39, 33], 1, 1, 3) s  R2ThermalI=repmat([.0109, .0029, .0013; .0069, .0024, .0012; .0047, .0026, .0013; .0034, .0016, .001; .0033, .0023, .0014; .0033, .0018, .0011; .0028, .0017, .0011], 1, 1, 3) Ohm  Tau2ThermalI=repmat([20, 36, 39; 31, 45, 39; 109, 105, 61; 36, 29, 26; 59, 77, 67; 40, 33, 29; 25, 39, 33], 1, 1, 3) s  R3ThermalI=repmat([.0109, .0029, .0013; .0069, .0024, .0012; .0047, .0026, .0013; .0034, .0016, .001; .0033, .0023, .0014; .0033, .0018, .0011; .0028, .0017, .0011], 1, 1, 3) Ohm  Tau3ThermalI=repmat([20, 36, 39; 31, 45, 39; 109, 105, 61; 36, 29, 26; 59, 77, 67; 40, 33, 29; 25, 39, 33], 1, 1, 3) s  DischargeR1Thermal=[.0109, .0029, .0013; .0069, .0024, .0012; .0047, .0026, .0013; .0034, .0016, .001; .0033, .0023, .0014; .0033, .0018, .0011; .0028, .0017, .0011] Ohm  DischargeTau1Thermal=[20, 36, 39; 31, 45, 39; 109, 105, 61; 36, 29, 26; 59, 77, 67; 40, 33, 29; 25, 39, 33] s  ChargeR1Thermal=[.0109, .0029, .0013; .0069, .0024, .0012; .0047, .0026, .0013; .0034, .0016, .001; .0033, .0023, .0014; .0033, .0018, .0011; .0028, .0017, .0011] Ohm  ChargeTau1Thermal=[20, 36, 39; 31, 45, 39; 109, 105, 61; 36, 29, 26; 59, 77, 67; 40, 33, 29; 25, 39, 33] s  DischargeR2Thermal=[.0109, .0029, .0013; .0069, .0024, .0012; .0047, .0026, .0013; .0034, .0016, .001; .0033, .0023, .0014; .0033, .0018, .0011; .0028, .0017, .0011] Ohm  DischargeTau2Thermal=[20, 36, 39; 31, 45, 39; 109, 105, 61; 36, 29, 26; 59, 77, 67; 40, 33, 29; 25, 39, 33] s  ChargeR2Thermal=[.0109, .0029, .0013; .0069, .0024, .0012; .0047, .0026, .0013; .0034, .0016, .001; .0033, .0023, .0014; .0033, .0018, .0011; .0028, .0017, .0011] Ohm  ChargeTau2Thermal=[20, 36, 39; 31, 45, 39; 109, 105, 61; 36, 29, 26; 59, 77, 67; 40, 33, 29; 25, 39, 33] s  DischargeR3Thermal=[.0109, .0029, .0013; .0069, .0024, .0012; .0047, .0026, .0013; .0034, .0016, .001; .0033, .0023, .0014; .0033, .0018, .0011; .0028, .0017, .0011] Ohm  DischargeTau3Thermal=[20, 36, 39; 31, 45, 39; 109, 105, 61; 36, 29, 26; 59, 77, 67; 40, 33, 29; 25, 39, 33] s  ChargeR3Thermal=[.0109, .0029, .0013; .0069, .0024, .0012; .0047, .0026, .0013; .0034, .0016, .001; .0033, .0023, .0014; .0033, .0018, .0011; .0028, .0017, .0011] Ohm  ChargeTau3Thermal=[20, 36, 39; 31, 45, 39; 109, 105, 61; 36, 29, 26; 59, 77, 67; 40, 33, 29; 25, 39, 33] s  SelfDischargeResistor=simscape.battery.enum.cells.BatteryEnable.Disabled  SelfDischargeR=7e3 Ohm  SelfDischargeRThermal=[8000, 7000, 6000] Ohm  CyclingAgingMethod=simscape.battery.enum.cells.CyclingAgingMethod.disabled  CycleCalculationMethod=simscape.battery.enum.cells.CycleCalculationMethod.EquivalentCycles  NumDisCycles=100  OCVChange=0  R0Change=0  CapacityChange=0  SelfDischargeRChange=0  R1Change=0  R2Change=0  R3Change=0  NumDisCyclesBreakpoints=[0, 100, 200, 300]  AgingTemperatureBreakpoints=[298.15, 323.15] K  AgingCurrentBreakpoints=[-.1, -.5, -5] A  OCVChangeVec=[0, 0, 0, 0]  OCVChangeThermal=[0, 0; 0, 0; 0, 0; 0, 0]  R0ChangeVec=[0, 0, 0, 0]  R0ChangeThermal=[0, 0; 0, 0; 0, 0; 0, 0]  R0ChangeThermalI=repmat(0, 4, 2, 3)  R0CyclingChangeInitialTarget=0  CapacityChangeVec=[0, 0, 0, 0]  CapacityChangeThermal=[0, 0; 0, 0; 0, 0; 0, 0]  CapacityChangeThermalI=repmat(0, 4, 2, 3)  CapacityCyclingChangeInitialTarget=0  SelfDischargeRChangeVec=[0, 0, 0, 0]  SelfDischargeRChangeThermal=[0, 0; 0, 0; 0, 0; 0, 0]  SelfDischargeRChangeThermalI=repmat(0, 4, 2, 3)  SelfDischargeRCyclingChangeInitialTarget=0  R1ChangeVec=[0, 0, 0, 0]  R1ChangeThermal=[0, 0; 0, 0; 0, 0; 0, 0]  R1ChangeThermalI=repmat(0, 4, 2, 3)  R1CyclingChangeInitialTarget=0  R2ChangeVec=[0, 0, 0, 0]  R2ChangeThermal=[0, 0; 0, 0; 0, 0; 0, 0]  R2ChangeThermalI=repmat(0, 4, 2, 3)  R2CyclingChangeInitialTarget=0  R3ChangeVec=[0, 0, 0, 0]  R3ChangeThermal=[0, 0; 0, 0; 0, 0; 0, 0]  R3ChangeThermalI=repmat(0, 4, 2, 3)  R3CyclingChangeInitialTarget=0  CalendarAgeResistance=simscape.battery.enum.cells.BatteryEnable.Disabled  CalendarAgeCapacity=simscape.battery.enum.cells.BatteryEnable.Disabled  CalendarAgingMethod=simscape.battery.enum.cells.CalendarAgingMethod.equation  StorageVariable=simscape.battery.enum.cells.StorageVariable.OCV  OCVDuringStorage=0.9  SOCDuringStorage=0.6  StorageTimeIntervals=[0] d  StorageTemperatures=[273] K  ResistanceScalingOCV=2.2134e6  ResistanceScalingOCVOffset=1.632e6  ResistanceExponentialIncrease=0.515833569 V  ResistanceTimeExponent=0.75  ResistanceAgeTemperatureBreakpoints=[273.15, 298.15, 323.15] K  ResistanceAgeTimeBreakpoints=[0, 90, 180, 270] d  PercentResistanceChange=[0, 0, 0]  ResistanceTimeBreakpoints=100 d  PercentResistanceChangeThermal=[0, 0, 0; 0, 0, 0; 0, 0, 0; 0, 0, 0]  CapacityScalingOCV=1.5097e07  CapacityScalingOCVOffset=8.3625e06  CapacityExponentialIncrease=0.6011 V  CapacityTimeExponent=0.75  CapacityAgeTemperatureBreakpoints=[273.15, 298.15, 323.15] K  CapacityAgeTimeBreakpoints=[0, 90, 180, 270] d  PercentCapacityChange=[0, 0, 0]  CapacityTimeBreakpoints=100 d  PercentCapacityChangeThermal=[0, 0, 0; 0, 0, 0; 0, 0, 0; 0, 0, 0]  SimulationTemperature=298.15 K  BatteryThermalMass=100 J/K  NumThermalModels=6  ThermalConductivityZ=18 W/(K*m)  CrossSectionalAreaXY=3.5e-4 m^2  Height=0.07 m  ReversibleHeatModel=simscape.battery.enum.cells.ReversibleHeatModel.Disabled  EntropicCoefficient=[0, 0, 0, 0, 0, 0, 0] mV/K  CurrentDirectionality=simscape.battery.enum.cells.BatteryEnable.Disabled  stateOfCharge_specify=on  stateOfCharge_priority=High  stateOfCharge=B  stateOfCharge_nominal_specify=off  stateOfCharge_nominal_value=1  stateOfCharge_nominal_unit=1  batteryVoltage_specify=off  batteryVoltage_priority=None  batteryVoltage=0 V  batteryVoltage_nominal_specify=off  batteryVoltage_nominal_value=1  batteryVoltage_nominal_unit=V  batteryCurrent_specify=off  batteryCurrent_priority=None  batteryCurrent=0 A  batteryCurrent_nominal_specify=off  batteryCurrent_nominal_value=1  batteryCurrent_nominal_unit=A  numCycles_specify=off  numCycles_priority=High  numCycles=0  numCycles_nominal_specify=off  numCycles_nominal_value=1  numCycles_nominal_unit=1  batteryTemperature_specify=off  batteryTemperature_priority=High  batteryTemperature=298.15 K  batteryTemperature_nominal_specify=off  batteryTemperature_nominal_value=1  batteryTemperature_nominal_unit=K  hysteresisState_specify=off  hysteresisState_priority=High  hysteresisState=0  hysteresisState_nominal_specify=off  hysteresisState_nominal_value=1  hysteresisState_nominal_unit=1  isExothermFaulted_specify=off  isExothermFaulted_priority=None  isExothermFaulted=0  isExothermFaulted_nominal_specify=off  isExothermFaulted_nominal_value=1  isExothermFaulted_nominal_unit=1  reactionHeatRate_specify=off  reactionHeatRate_priority=None  reactionHeatRate=0 W  reactionHeatRate_nominal_specify=off  reactionHeatRate_nominal_value=1  reactionHeatRate_nominal_unit=W  reactionExtent_specify=off  reactionExtent_priority=None  reactionExtent=0  reactionExtent_nominal_specify=off  reactionExtent_nominal_value=1  reactionExtent_nominal_unit=1  shortResistorPower_specify=off  shortResistorPower_priority=None  shortResistorPower=0 W  shortResistorPower_nominal_specify=off  shortResistorPower_nominal_value=1  shortResistorPower_nominal_unit=W
      | [
      |     2.50  2.51  2.52
      |     2.78  2.79  2.80
      |     3.07  3.08  3.09
      |     3.35  3.36  3.37
      |     3.63  3.64  3.65
      |     3.91  3.92  3.93
      |     4.20  4.21  4.22
      | ]
      |  V
  Current Sensor1 : fl_lib/Electrical/Electrical Sensors/Current Sensor
  Current Sensor3 : fl_lib/Electrical/Electrical Sensors/Current Sensor
  PS-Simulink Converter2 : nesl_utility/PS-Simulink Converter  PhysicalDomain=network_engine_domain  SubClassName=ps_output  LeftPortType=input  RightPortType=output  PseudoPeriodic=off  Frequencies=[]  VectorFormat=inherit  Unit=inherit  AffineConversion=off
  PS-Simulink Converter4 : nesl_utility/PS-Simulink Converter  PhysicalDomain=network_engine_domain  SubClassName=ps_output  LeftPortType=input  RightPortType=output  PseudoPeriodic=off  Frequencies=[]  VectorFormat=inherit  Unit=inherit  AffineConversion=off
  PS-Simulink Converter6 : nesl_utility/PS-Simulink Converter  PhysicalDomain=network_engine_domain  SubClassName=ps_output  LeftPortType=input  RightPortType=output  PseudoPeriodic=off  Frequencies=[]  VectorFormat=inherit  Unit=inherit  AffineConversion=off
  Resistor1 : fl_lib/Electrical/Electrical Elements/Resistor  R=R Ohm  i_specify=off  i_priority=None  i=0 A  i_nominal_specify=off  i_nominal_value=1  i_nominal_unit=A  v_specify=off  v_priority=None  v=0 V  v_nominal_specify=off  v_nominal_value=1  v_nominal_unit=V
  Voltage Sensor1 : fl_lib/Electrical/Electrical Sensors/Voltage Sensor
  thermal : PMIOPort  Side=Left
  input : PMIOPort  Port=2  Side=Left
  output : PMIOPort  Port=3  Side=Right
  RC2 : Outport
  BC2 : Outport  Port=2
  V2 : Outport  Port=3
  wires:
  PS-Simulink Converter2/1 -> V2/1
  PS-Simulink Converter4/1 -> RC2/1
  PS-Simulink Converter6/1 -> BC2/1
  connections:
  Battery Equivalent Circuit1/RConn2 -- thermal/RConn1
  Resistor1/RConn1 -- Voltage Sensor1/RConn2 -- output/RConn1 -- Battery Equivalent Circuit1/RConn1
  Current Sensor1/LConn1 -- Current Sensor3/LConn1 -- Voltage Sensor1/LConn1 -- input/RConn1
  Voltage Sensor1/RConn1 -- PS-Simulink Converter2/LConn1
  Current Sensor1/RConn2 -- Resistor1/LConn1
  Current Sensor3/RConn2 -- Battery Equivalent Circuit1/LConn1
  Current Sensor3/RConn1 -- PS-Simulink Converter6/LConn1
  Current Sensor1/RConn1 -- PS-Simulink Converter4/LConn1
